simulink model "FULL_SIM_BUILDUP"  (R2025b)
settings: Solver=VariableStepAuto  StartTime=0.0  StopTime=10.0  RelTol=1e-3
InitFcn:
  | %% State Estimator
  | p_init  = [0,0,0];
  | v_init  = [0,0,0];
  | q_init  = [1,0,0,0];
  | bg_init = [1.045715,0.002947,-0.517855];
  | ba_high_init = [-7.395250,-4.820243,-18.177021];
  | ba_low_init = [-0.021725, 0.062643, -0.022747];
  | 
  | taug_init = [1.105; 1.105; 1.105];
  | taua_high_init = [8.731; 8.731; 8.731];
  | qg_init = [4.390573e-05; 2.319960e-05; 1.494807e-05];
  | qa_high_init = [8.774166e-04; 7.720775e-04; 1.336849e-03];
  | 
  | x_init = [p_init, v_init, q_init, bg_init, ba_high_init, ba_low_init]';
  | P_init = zeros(19);
  | dt = 1/1000;
  | %% Sensors
  | % Low-g accelerometer
  | dt_lowaccel = 1/120;
  | ba_low_init = [-0.021725; 0.062643; -0.022747];
  | taua_low = [1.437; 1.437; 1.437];
  | qa_low = [1.483796e-6; 1.224280e-6; 1.983171e-6];
  | noise_std_lowaccel = [0.020005; 0.021677; 0.025995];
  | quant_step_lowaccel = 0.004905;
  | 
  | % Gyro
  | dt_gyro = 1/120;
  | gyro_bias_init = [1.045715; 0.002947; -0.517855];
  | gyro_tau = [1.105; 1.105; 1.105];
  | gyro_drift_variance = [4.390573e-5; 2.319960e-5; 1.494807e-5];
  | gyro_noise_std = [0.130937; 0.093580; 0.075444];
  | gyro_quant_step = 0.05;
  | 
  | % High-g acceleromter
  | dt_highaccel = 1/120;
  | highaccel_bias_init = [-7.395250; -4.820243; -18.177021];
  | highaccel_tau = [8.731; 8.731; 8.731];
  | highaccel_drift_variance = [8.774166e-4; 7.720775e-4; 1.336849e-3];
  | highaccel_noise_std = [1.645664; 1.487596; 1.836378];
  | highaccel_quant_step = 0.5;
  | 
  | % Barometer [K Pa]
  | dt_baro = 1/50;
  | baro_bias_init = [0; 0];
  | baro_tau = [11.9906; 88.5141];
  | baro_drift_variance = [4.1889e-8; 2.9560e-4];
  | baro_noise_std = [0.01; 0.35];
  | baro_quant_step = [0.01; 0.06];
  | 
  | % Magnetometer
  | dt_mag = 1/50;
  | mag_calibration_offset = [-0.0705; -0.1152; 0.0250];
  | mag_calibration_matrix = [2.2439, -0.0154, -0.0144; -0.0154, 2.2042, -0.0970; -0.0144, -0.0097, 2.4001];
  | mag_bias_init = [0; 0; 0];
  | mag_tau = [6.9630; 7.8914; 6.3777];
  | mag_drift_variance = [1.1384e-11; 2.9369e-11; 4.0735e-11];
  | mag_noise_std = [1.2; 1.2; 1.2];
  | mag_quant_step = [0.0625; 0.0625; 0.0625];
  | 
  | % GPS
  | dt_gps = 1/50;
  | gps_bias_init = [0; 0; 0; 0; 0; 0; 0; 0; 0];
  | gps_tau = [116.2031; 204.0083; 88.1618; 0.3353; 1.4466; 0.8506; inf; inf; inf];
  | gps_drift_variance = [6.1178e-20; 7.8958e-20; 1.0101e-2; 1.1742e-4; 6.3880e-5; 9.5787e-5; 0; 0; 0];
  | gps_noise_std = [1.35e-7; 1.35e-7; 1.35e-8; 5e-5; 5e-5; 5e-5; 0; 0; 0];
  | gps_quant_step = [0.5e-7; 0.5e-7; 5e-4; 5e-4; 5e-4; 5e-4; 1; 1; 0.1];
  | 
  | % LiDAR
  | dt_lidar = 1/50;
  | lidar_bias_init = 0.01;
  | lidar_tau = 120;
  | lidar_drift_variance = 1e-6;
  | lidar_noise_std = 0.03;
  | lidar_quant_step = 0.01;
  | lidar_min_range = 0.2;
  | lidar_max_range = 8.0;
settings Model: Creator=Admin  LastModifiedBy=Admin

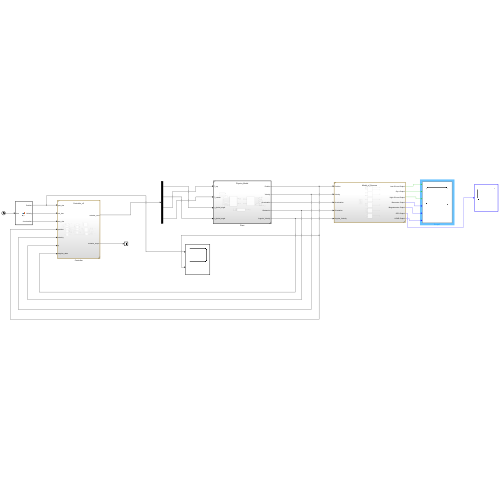
[thumbnail: Simulink's stored preview of the top-level diagram]
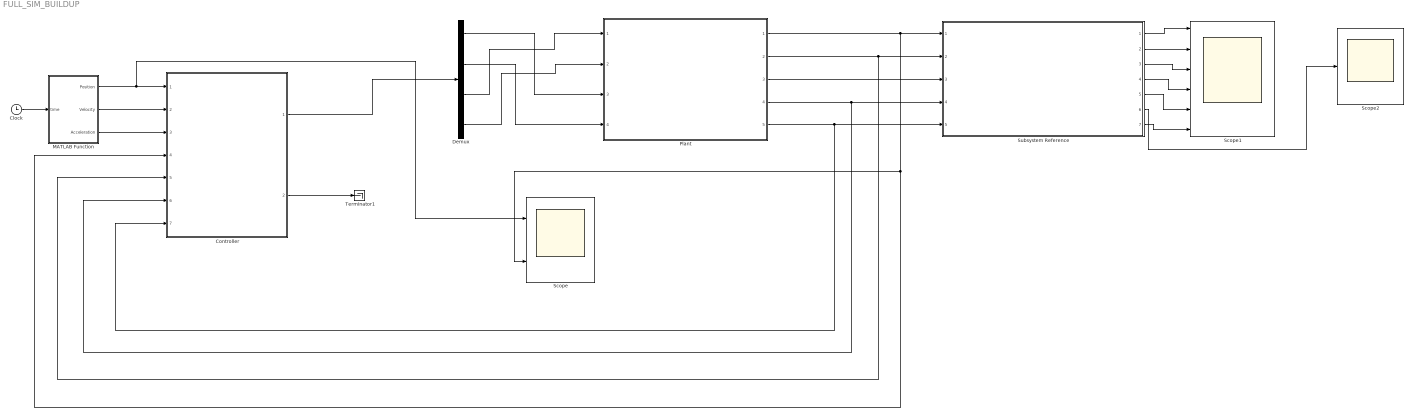
== system FULL_SIM_BUILDUP ==
  Clock : Clock
  Controller : Subsystem  ReferencedSubsystem=Controller_v2
  Demux : Demux
  MATLAB Function : MATLAB Function  TreatAsAtomicUnit=on
  Plant : Subsystem  ReferencedSubsystem=Physics_Model
  Scope : Scope  NumInputPorts=2
      settings: ActiveDisplayYMinimum=-0.998275528438487  ActiveDisplayYMaximum=6.0632194159063513
  Scope1 : Scope  NumInputPorts=6
      settings: ActiveDisplayYMinimum=-3.0257718749999993  ActiveDisplayYMaximum=13.203646874999999
  Scope2 : Scope
      settings: ActiveDisplayYMinimum=-11.251252281249997  ActiveDisplayYMaximum=58.47127053125  DataLoggingVariableName=ScopeData6
  Subsystem Reference : Subsystem  ReferencedSubsystem=Model_of_Sensors
  Terminator1 : Terminator
  wires:
  Demux/4 -> Plant/2
  Demux/2 -> Plant/4
  Demux/1 -> Plant/3
  Demux/3 -> Plant/1
  Clock/1 -> MATLAB Function/1(time)
  Controller/1 -> Demux/1
  MATLAB Function/1(Position) -> Scope/1, Controller/1
  MATLAB Function/2(Velocity) -> Controller/2
  MATLAB Function/3(Acceleration) -> Controller/3
  Controller/2 -> Terminator1/1
  Plant/1 -> Scope/2, Controller/4, Subsystem Reference/1
  Plant/4 -> Subsystem Reference/4, Controller/6
  Plant/5 -> Subsystem Reference/5, Controller/7
  Plant/2 -> Controller/5, Subsystem Reference/2
  Plant/3 -> Subsystem Reference/3
  Subsystem Reference/1 -> Scope1/1
  Subsystem Reference/2 -> Scope1/2
  Subsystem Reference/3 -> Scope1/3
  Subsystem Reference/4 -> Scope1/4
  Subsystem Reference/5 -> Scope1/5
  Subsystem Reference/7 -> Scope1/6
  Subsystem Reference/6 -> Scope2/1

== matlab function FULL_SIM_BUILDUP/MATLAB Function ==
  data: time input; Position output; Velocity output; Acceleration output
function [Position, Velocity, Acceleration] = fcn(time)
% Frames:
% - Position, Velocity, Acceleration in NED
% - Quaternion scalar-first [q0; q1; q2; q3]
% - Angular_Velocity = [p; q; r] in rad/s

% -----------------------------
% Trajectory configuration
% -----------------------------
T.x0 = 0;
T.xi = 5;
T.xf = 0;

T.y0 = 0;
T.yi = 5;
T.yf = 0;

T.z0 = 0;
T.zi = -5;
T.zf = 0;

T.t1       = 5.0;
T.t2       = 5.0;
T.dt_blend = 2.0;
T.frac_tb  = 0.20;
T.useStep  = false;

% -----------------------------
% Translational motion
% -----------------------------
[Position, Velocity, Acceleration] = trapezoidalRefBlockXYZ(time, T);
% Position = [0;0;0];
% Velocity = [0;0;0];
% Acceleration = [0;0;0];
